simulink model "FSEA_Vehicle"  (R2026a)
settings: Solver=ode23tb  StopTime=5  FixedStep=.001  RelTol=1e-1
model workspace (MAT data in the model file):
  A_mu = 10
  B_reff = 8.386
  CONVERTER_DATA = [0  137.465208994  2.232; 0.1  137.065019157  2.075; 0.2  135.864449646  1.975; 0.3  135.664354728  1.846; 0.4  137.565256453  1.72; 0.5  140.366585312  1.564; 0.6  145.268910814  1.409; 0.7  152.872517717  1.254; 0.8  162.9773111  1.096; 0.81  164.27792807  1.08; 0.82  166.178829795  1.061; 0.83  167.979684062  1.043; 0.84  170.080680706  1.028; 0.85  172.781962105  1.012; 0.86  175.383196045  1.002; 0.87  179.585189333  1.002; 0.88  183.587087703  1.001; 0.89  189.890077635  0.998; 0.9  197.693779455  0.999; 0.92  215.902417037  1.001; 0.94  244.515990379  1.002]
  Cps = 2
  Cz = 7766.25
  DOWN_TABLE = [0  5  10  20  30; 0  5  10  20  30; 0  7.5  20  30  40; 0  7.5  20  30  40; 0  15  30  50  60; 0  15  30  50  60]
  DOWN_TH_BP = [0 5 40 50 90 100]
  D_reff = 0.25826
  EMAP = [-40  -44  -49  -53  -57  -61  -65  -70  -74  -78  -82; 215  117  85  66  44  29  10  -2  -13  -22  -32; 245  208  178  148  122  104  85  66  48  33  18; 264  260  241  219  193  167  152  133  119  96  85; 264  279  282  275  260  238  223  208  189  171  152; 267  290  293  297  290  275  260  256  234  212  193; 267  297  305  305  305  301  293  282  267  249  226; 267  301  308  312  319  323  319  316  297  279  253; 267  301  312  319  327  327  327  327  312  293  267; 267  301  312  319  327  334  334  334  319  305  275]
  F0z = [6086.4 4324.8]
  F_reff = 0.07394
  F_zmax = 10000
  F_zmin = 100
  F_zo = 4000
  Kz = 48000
  MF.f.mu_x = 1.2
  MF.f.mu_y = 0.935
  MF.f.Bx = 11.7
  MF.f.By = 8.86
  MF.f.Cx = 1.69
  MF.f.Cy = 1.19
  MF.f.Ex = 0.377
  MF.f.Ey = -1.21
  MF.f.Cxalpha = 1.09
  MF.f.Cykappa = 1.08
  MF.f.Bx1 = 12.4
  MF.f.Bx2 = -10.8
  MF.f.By1 = 6.46
  MF.f.By2 = 4.2
  MF.f.Sh = 0
  MF.f.Sv = 0
  MF.r.mu_x = 1.2
  MF.r.mu_y = 0.961
  MF.r.Bx = 11.1
  MF.r.By = 9.3
  MF.r.Cx = 1.69
  MF.r.Cy = 1.19
  MF.r.Ex = 0.362
  MF.r.Ey = -1.11
  MF.r.Cxalpha = 1.09
  MF.r.Cykappa = 1.08
  MF.r.Bx1 = 12.4
  MF.r.Bx2 = -10.8
  MF.r.By1 = 6.46
  MF.r.By2 = 4.2
  MF.r.Sh = 0
  MF.r.Sv = 0
  NCyl = 6
  NE_VEC = [800 1200 1600 2000 2400 2800 3200 3600 4000 4400 4800]
  Pstd = 101325
  Rair = 287
  SUS.Stiffness = 24000
  SUS.Damping.Constant = 1262
  SUS.Damping.Rebound = [4040 4950 2883 2043]
  SUS.Damping.Compression = [3600 3420 1863 1472]
  SUS.PistonSpeed = [0.05 0.1 0.3 0.6]
  SUS.UnsprungMass.Fr = 21.0693333333
  SUS.UnsprungMass.Rr = 21.0693333333
  TH_VEC = [0; 20; 30; 40; 50; 60; 70; 80; 90; 100]
  TWAITdn = 1.25
  TWAITup = 0.1
  Tin = [1  2; 2  2; 3  2; 4  2; 5  2; 6  0; 7  0; 8  0; 9  0; 10  0]
  Tstd = 293.15
  UP_TABLE = [7.5  25  40  50  60; 7.5  25  40  50  60; 15  35  50  60  70; 25  45  60  70  80; 40  70  90  100  110; 40  80  90  100  110]
  UP_TH_BP = [0 25 35 50 90 100]
  VEH.Mass = 1181
  VEH.StaticNormalFrontLoad.FR = 264.666666667
  VEH.StaticNormalFrontLoad.FL = 264.666666667
  VEH.StaticNormalRearLoad.RR = 322
  VEH.StaticNormalRearLoad.RL = 322
  VEH.WheelBase = 3.075
  VEH.FrontAxlePositionfromCG = 1.515
  VEH.RearAxlePositionfromCG = 1.504
  VEH.HeightCG = 0.134
  VEH.FrontalArea = 2.11
  VEH.DragCoefficient = 0.33
  VEH.NumberOfWheelsPerAxle = 2
  VEH.PitchMomentInertia = 1922.66666667
  VEH.RollMomentInertia = 432.333333333
  VEH.YawMomentInertia = 2066
  VEH.SteeringRatio = 18
  VEH.TrackWidth = 1.922
  VEH.SprungMass = 1096.72266667
  VEH.InitialLongPosition = 0
  VEH.InitialLatPosition = 0
  VEH.InitialVertPosition = 0
  VEH.InitialRollAngle = 0
  VEH.InitialPitchAngle = 0
  VEH.InitialYawAngle = 0
  VEH.InitialLongVel = 0
  VEH.InitialLatVel = 0
  VEH.InitialVertVel = 0
  VEH.InitialRollRate = 0
  VEH.InitialPitchRate = 0
  VEH.InitialYawRate = 0
  VEH.UnsprungMassRearAxle = 160
  VEH.UnsprungMassFrontAxle = 100
  V_o = 16.7
  V_xlow = 1
  Vd = 0.00346
  WH.Tire.Radius.Front = 0.384
  WH.Tire.Radius.Rear = 0.401
  WH.Tire.Sidewall = 0.245
  WH.Tire.RollingResistCoeff = 0.0103
  WH.Tire.Magic.B = 10
  WH.Tire.Magic.C = 1.9
  WH.Tire.Magic.D = 1
  WH.Tire.Magic.E = 0.97
  WH.Tire.Magic.Bx = 12
  WH.Tire.Magic.Cx = 1.9
  WH.Tire.Magic.Dx = 0.72
  WH.Tire.Magic.Ex = 0.95
  WH.Tire.Magic.By = 12
  WH.Tire.Magic.Cy = 1.3
  WH.Tire.Magic.Dy = 0.75
  WH.Tire.Magic.Ey = 0.2
  WH.Tire.Front.Ky = 40000
  WH.Tire.Rear.Ky = 40000
  WH.Tire.Kz = 320000
  WH.Tire.Damping = 100
  WH.Inertia = 1.00333333333
  WH.Mass = 11.4333333333
  WH.DampingCoefficient = 0.01
  WH.VelocityTol = 0.1
  a = 1.515
  alpha_max = 1.5
  alpha_min = -1.5
  b = 1.504
  c_zo = 209651
  epsilon = 0.1
  f_air = [0 0 0 0 0 0 0 0 0 0 0 0 ... (256 elements, 16x16)]
  f_co = [0 0 0 0 0 0 0 0 0 0 0 0 ... (256 elements, 16x16)]
  f_co2 = [0 0 0 0 0 0 0 0 0 0 0 0 ... (256 elements, 16x16)]
  f_eff = [352.135682859 352.135682859 320.724378192 303.655312657 295.930136708 291.240087194 291.240271258 291.240312459 291.240275452 291.240198499 291.240100781 291.240018769 ... (256 elements, 16x16)]
  f_fuel = [0 0 0 0 0 0 0 0 0 0 0 0 ... (256 elements, 16x16)]
  f_hc = [0 0 0 0 0 0 0 0 0 0 0 0 ... (256 elements, 16x16)]
  f_nox = [0 0 0 0 0 0 0 0 0 0 0 0 ... (256 elements, 16x16)]
  f_pm = [0  0  0  0  0  0  0  0  0  0  0  0  0  0  0  0; 0  0  0  0  0  0  0  0  0  0  0  0  0  0  0  0; 0  0  0  0  0  0  0  0  0  0  0  0  0  0  0  0; 0  0  0  0  0  0  0  0  0  0  0  0  0  0  0  0; 0  0  0  0  0  0  0  0  0  0  0  0  0  0  0  0; 0  0  0  0  0  0  0  0  0  0  0  0  0  0  0  0; 0  0  0  0  0  0  0  0  0  0  0  0  0  0  0  0; 0  0  0  0  0  0  0  0  0  0  0  0  0  0  0  0; 0  0  0  0  0  0  0  0  0  0  0  0  0  0  0  0; 0  0  0  0  0  0  0  0  0  0  0  0  0  0  0  0; 0  0  0  0  0  0  0  0  0  0  0  0  0  0  0  0; 0  0  0  0  0  0  0  0  0  0  0  0  0  0  0  0; 0  0  0  0  0  0  0  0  0  0  0  0  0  0  0  0; 0  0  0  0  0  0  0  0  0  0  0  0  0  0  0  0; 0  0  0  0  0  0  0  0  0  0  0  0  0  0  0  0; 0  0  0  0  0  0  0  0  0  0  0  0  0  0  0  0]
  f_susp_axl_bp = [1 2]
  f_susp_dz_bp = [-4 -0.14 -0.13 -0.12 -0.11 -0.1 -0.09 -0.08 -0.07 -0.06 -0.05 -0.04 -0.03 -0.02 -0.01 0 0.01 0.02 0.03 0.04 0.05 0.06 0.07 0.08 0.09 0.1 0.11 0.12 0.13 0.14 4]
  f_susp_dzdot_bp = [-4 -0.14 -0.13 -0.12 -0.11 -0.1 -0.09 -0.08 -0.07 -0.06 -0.05 -0.04 -0.03 -0.02 -0.01 0 0.01 0.02 0.03 0.04 0.05 0.06 0.07 0.08 0.09 0.1 0.11 0.12 0.13 0.14 4]
  f_susp_fmz = [-213379.591456 -28099.591456 -27619.591456 -27139.591456 -26659.591456 -26179.591456 -25699.591456 -25219.591456 -24739.591456 -24259.591456 -23779.591456 -23299.591456 ... (468968 elements, 31x31x61x2x4)]
  f_susp_geom = [-0.832564012244 0.043269987756 0.045538987756 0.047807987756 0.050076987756 0.052345987756 0.054614987756 0.056883987756 0.059152987756 0.061421987756 0.063690987756 0.065959987756 ... (11346 elements, 31x61x2x3)]
  f_susp_strgdelta_bp = [-0.523598775598 -0.506145483078 -0.488692190558 -0.471238898038 -0.453785605519 -0.436332312999 -0.418879020479 -0.401425727959 -0.383972435439 -0.366519142919 -0.349065850399 -0.331612557879 -0.314159265359 -0.296705972839 -0.279252680319 -0.261799387799 -0.244346095279 -0.226892802759 -0.209439510239 -0.191986217719 -0.174532925199 -0.157079632679 -0.13962634016 -0.12217304764 -0.10471975512 -0.0872664625997 -0.0698131700798 -0.0523598775598 -0.0349065850399 -0.0174532925199 0 0.0174532925199 0.0349065850399 0.0523598775598 0.0698131700798 0.0872664625997 0.10471975512 0.12217304764 0.13962634016 0.157079632679 0.174532925199 0.191986217719 0.209439510239 0.226892802759 0.244346095279 0.261799387799 0.279252680319 0.296705972839 0.314159265359 0.331612557879 0.349065850399 0.366519142919 0.383972435439 0.401425727959 0.418879020479 0.436332312999 0.453785605519 0.471238898038 0.488692190558 0.506145483078 0.523598775598]
  f_tbrake = [0 76.8593923996 105.140482948 131.533638111 157.926793274 176.658631717 176.65727296 176.656856686 176.656879077 176.657093756 176.657404516 176.65772406 ... (256 elements, 16x16)]
  f_tbrake_n_bpt = [0 649.519052838 912.419621844 1175.32019085 1438.22075986 1701.12132886 1964.02189787 2226.92246687 2489.82303588 2752.72360489 3015.62417389 3278.5247429 3541.4253119 3804.32588091 4067.22644992 4330.12701892]
  f_tbrake_t_bpt = [0 34.6410161514 61.0341713143 87.4273264773 113.82048164 140.213636803 166.606791966 192.999947129 219.393102292 245.786257455 272.179412618 298.572567781 324.965722944 351.358878107 377.75203327 404.145188433]
  f_texh = [766.752464599 766.752464599 786.17542386 801.679939032 884.591982581 910.574397722 910.571871054 910.570774534 910.570601632 910.570821151 910.571247242 910.571639815 ... (256 elements, 16x16)]
  f_twc_eff_co = [0.17 0.25 0.45 0.99 0.99 0.99 0.99]
  f_twc_eff_hc = [0.21 0.375 0.75 0.98 0.98 0.98 0.98]
  f_twc_eff_lam = [0.909090909 0.944055944 0.979020979 1 1.013986014 1.048951049 1.083916084]
  f_twc_eff_nox = [0.98 0.98 0.98 0.97 0.05 0.02 0]
  h = 0.134
  k_z = 50
  kappa_max = 1.5
  kappa_min = -1.5
  lam_Cx = 1
  lam_Cy = 1
  lam_Cz = 1
  lam_Ex = 1
  lam_Ey = 1
  lam_F_zo = 1
  lam_Hx = 1
  lam_Hy = 1
  lam_Kxkappa = 1
  lam_Kyalpha = 1
  lam_Kygamma = 1
  lam_Kzgamma = 1
  lam_Mr = 1
  lam_Mx = 1
  lam_My = 1
  lam_S = 1
  lam_VMx = 1
  lam_Vx = 1
  lam_Vy = 1
  lam_Vykappa = 1
  lam_muV = 0
  lam_mux = 1
  lam_muy = 1
  lam_t = 1
  lam_xalpha = 1
  lam_ykappa = 1
  numWheel = 4
  p_Cx1 = 1.579
  p_Cy1 = 1.3332
  p_Dx1 = 1.0422
  p_Dx2 = -0.08285
  p_Dx3 = 0
  p_Dy1 = 0.8784
  p_Dy2 = -0.06445
  p_Dy3 = 0
  p_Ex1 = 0.11185
  p_Ex2 = 0.3127
  p_Ex3 = 0
  p_Ex4 = 0.001603
  p_Ey1 = -0.8227
  p_Ey2 = -0.6062
  p_Ey3 = 0.09825
  p_Ey4 = -6.546
  p_Ey5 = 0
  p_Fz1 = 0.7098
  p_Hx1 = 0.00021585
  p_Hx2 = 0.0011538
  p_Hy1 = -0.0018043
  p_Hy2 = 0.003518
  p_Kx1 = 21.69
  p_Kx2 = 13.774
  p_Kx3 = -0.4119
  p_Ky1 = -15.314
  p_Ky2 = 1.7044
  p_Ky3 = 0.36986
  p_Ky4 = 1.9896
  p_Ky5 = 0
  p_Ky6 = -0.9004
  p_Ky7 = -0.2328
  p_Vx1 = 1.5973e-05
  p_Vx2 = 0.0001043
  p_Vy1 = -0.006642
  p_Vy2 = 0.03597
  p_Vy3 = -0.1621
  p_Vy4 = -0.4908
  p_pmx1 = 0
  p_px1 = -0.3489
  p_px2 = 0.382
  p_px3 = -0.09634
  p_px4 = 0.06447
  p_py1 = -0.6249
  p_py2 = -0.06535
  p_py3 = -0.1668
  p_py4 = 0.2834
  p_py5 = 0
  path.ISO3888p2.x = [0 2 12 25.5 36.5 49 61]
  path.ISO3888p2.y = [0 0 0 3.725 3.725 0 0]
  path.ISO3888p2.ylb = [1.225 1.225 1.225 4.725 4.725 1.5 1.5]
  path.ISO3888p2.yrb = [-1.225 -1.225 -1.225 2.225 2.225 -1.5 -1.5]
  path.CUSC.x = [10.668 21.336 36.576 54.864 73.152]
  path.CUSC.y = [0 0 5.1816 0 0]
  path.CUSC.ylb = [1.2192 1.2192 7.0104 1.8288 1.8288]
  path.CUSC.yrb = [-1.2192 -1.2192 3.3528 -1.8288 -1.8288]
  pio = 220000
  q_Fcx = 0
  q_Fz2 = 15.4
  q_Fzy = 0
  q_reo = 0.9974
  q_sx1 = -0.007764
  q_sx10 = 0.2824
  q_sx11 = 5.349
  q_sx12 = 0
  q_sx13 = 0
  q_sx14 = 0
  q_sx2 = 1.1915
  q_sx3 = 0.013948
  q_sx4 = 4.912
  q_sx5 = 1.02
  q_sx6 = 22.83
  q_sx7 = 0.7104
  q_sx8 = -0.023393
  q_sx9 = 0.6581
  q_sy1 = 0.00702
  q_sy2 = 0
  q_sy3 = 0.001515
  q_sy4 = 8.514e-05
  q_sy5 = 0
  q_sy6 = 0
  q_sy7 = 0.9008
  q_sy8 = -0.4089
  q_v1 = 0.0007742
  q_v2 = 0.04667
  r_Bx1 = 12.531
  r_Bx2 = 9.532
  r_Bx3 = 0
  r_By1 = 10.615
  r_By2 = 7.705
  r_By3 = 3.433e-06
  r_By4 = 0
  r_Cx1 = 1.019
  r_Cy1 = 1.0585
  r_Ex1 = -0.4487
  r_Ex2 = -0.4726
  r_Ey1 = 0.3132
  r_Ey2 = 7.63e-06
  r_Hx1 = 0.0002374
  r_Hy1 = 0.011646
  r_Hy2 = 7.63e-06
  r_Vy1 = 0.05654
  r_Vy2 = 7.63e-06
  r_Vy3 = 0
  r_Vy4 = 99.9
  r_Vy5 = 2
  r_Vy6 = 15.814
  r_o = 0.3135
  reqTmaxT = [nan  nan  nan  nan  nan  nan  nan  nan; 0.285774810084  0.209689533834  0.17164689571  0.133604257585  0.0955616194602  nan  nan  nan; 0.647179872268  0.495009319769  0.41892404352  0.342838767271  0.266753491021  0.152625576647  nan  nan; nan  0.780329105704  0.66620119133  0.552073276956  0.437945362582  0.266753491021  0.152625576647  0.0955616194602; nan  nan  0.913478339141  0.761307786642  0.609137234143  0.380881405395  0.228710852897  0.152625576647; nan  nan  nan  0.970542296328  0.780329105704  0.495009319769  0.304796129146  0.209689533834; nan  nan  nan  nan  0.951520977265  0.609137234143  0.380881405395  0.266753491021; nan  nan  nan  nan  nan  0.723265148517  0.456966681645  0.323817448208; nan  nan  nan  nan  nan  0.837393062891  0.533051957894  0.380881405395; nan  nan  nan  nan  nan  0.951520977265  0.609137234143  0.437945362582; nan  nan  nan  nan  nan  nan  0.685222510393  0.495009319769; nan  nan  nan  nan  nan  nan  0.761307786642  0.552073276956; nan  nan  nan  nan  nan  nan  0.837393062891  0.609137234143; nan  nan  nan  nan  nan  nan  0.913478339141  0.66620119133; nan  nan  nan  nan  nan  nan  0.98956361539  0.723265148517; nan  nan  nan  nan  nan  nan  nan  0.780329105704; nan  nan  nan  nan  nan  nan  nan  0.837393062891; nan  nan  nan  nan  nan  nan  nan  0.894457020078; nan  nan  nan  nan  nan  nan  nan  0.951520977265; nan  nan  nan  nan  nan  nan  nan  nan; nan  nan  nan  nan  nan  nan  nan  nan]
  vehSpd = [0 2.77777777778 5.55555555556 8.33333333333 11.1111111111 13.8888888889 16.6666666667 19.4444444444 22.2222222222 25 27.7777777778 30.5555555556 33.3333333333 36.1111111111 38.8888888889 41.6666666667 44.4444444444 47.2222222222 50 52.7777777778 55.5555555556]
  vehWidth = 2
  w = 1
undefined symbols (not defined in the file or in its folder): InertFrm
libraries: sharedtransform x6, vehdynlibtirecommon x2, vehdynlibtire x2, autolibutils x2, autolibshared x2
(part 1 of 4)
settings Model: DataDictionary=PassVeh7DOF.sldd  ModifiedByFormat=The MathWorks, Inc.  SimulationMode=accelerator  Creator=The MathWorks, Inc.  LastModifiedBy=The MathWorks, Inc.
settings SolverCC: SolverJacobianMethodControl=FullPerturbation  ZeroCrossAlgorithm=Adaptive  DecoupledContinuousIntegration=on
settings DebuggingCC: ArtificialAlgebraicLoopMsg=none  MaskedZcDiagnostic=none  IgnoredZcDiagnostic=none  SignalLabelMismatchMsg=warning
settings ModelReferenceCC: ModelReferenceMinAlgLoopOccurrences=on

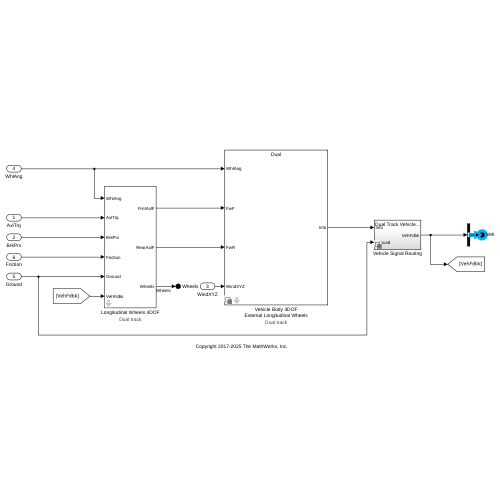
[thumbnail: Simulink's stored preview of the top-level diagram]
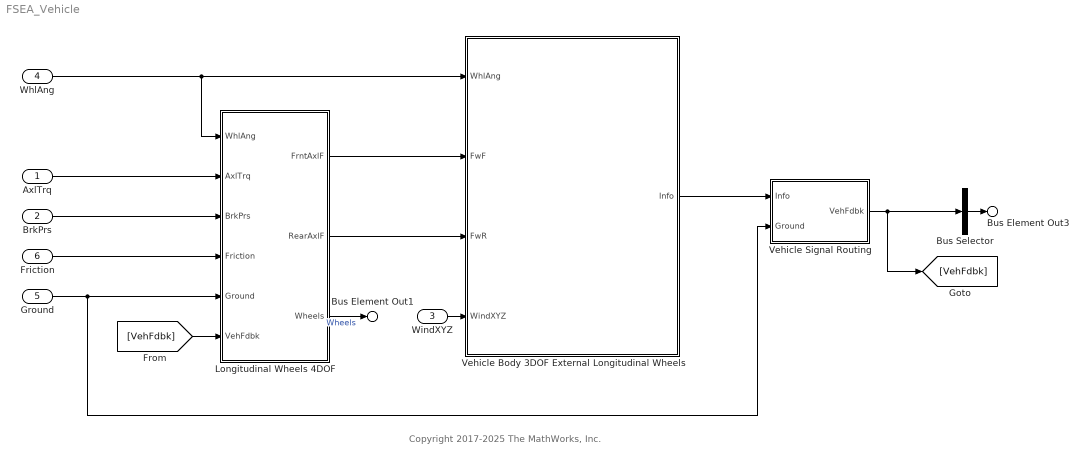
== system FSEA_Vehicle ==
  note: Copyright 2017-2025 The MathWorks, Inc.
  AxlTrq : Inport  Unit=N*m  PortDimensions=4
  BrkPrs : Inport  Port=2  Unit=Pa  PortDimensions=4
  WindXYZ : Inport  Port=3  PortDimensions=3
  WhlAng : Inport  Port=4  Unit=rad  PortDimensions=4
  Ground : Inport  Port=5  Unit=m  PortDimensions=4
  Friction : Inport  Port=6  Unit=1  PortDimensions=4
  Bus Selector : BusSelector  OutputSignals=InertFrm,BdyFrm  OutputAsBus=on
  Longitudinal Wheels 4DOF : Subsystem  VariantControl=1  mask{wheelMode=Dual track}
      mask prompts: wheelMode "Wheel mode:"
      settings: AttributesFormatString=%<wheelMode>
      mask TypeOptions wheelMode: Single track (bicycle) | Dual track
      mask Callback wheelMode:
      | switch get_param(gcb,'wheelMode')
      |     case 'Single track (bicycle)'
      |         set_param([bdroot '/Longitudinal Wheels 4DOF/Velocity and Vertical Load'],'OverrideUsingVariant','0')
      |         set_param([bdroot '/Longitudinal Wheels 4DOF/Axle Forces'],'OverrideUsingVariant','0')
      |     case 'Dual track'
      |         set_param([bdroot '/Longitudinal Wheels 4DOF/Velocity and Vertical Load'],'OverrideUsingVariant','1')
      |         set_param([bdroot '/Longitudinal Wheels 4DOF/Axle Forces'],'OverrideUsingVariant','1')
      |     otherwise
      |         set_param([bdroot '/Longitudinal Wheels 4DOF/Velocity and Vertical Load'],'OverrideUsingVariant','0')
      |         set_param([bdroot '/Longitudinal Wheels 4DOF/Axle Forces'],'OverrideUsingVariant','0')
      | end
  Vehicle Body 3DOF External Longitudinal Wheels : Subsystem  Variant=on  VariantControlMode=label  VariantControl=Variant1  LabelModeActiveChoice=1  mask(Example 3DOF vehicle model){trackMode=Dual track}
      mask prompts: trackMode "Vehicle Mode:"
      mask help: Select the variant of the 3DOF vehicle model. The wheel subsystem will be automatically configured accordingly.
      settings: AttributesFormatString=%<trackMode>
      mask TypeOptions trackMode: Single track (bicycle) | Dual track
      mask Callback trackMode:
      | switch get_param(gcb,'trackMode')
      |     case 'Single track (bicycle)'
      |         set_param([bdroot '/Vehicle Body 3DOF' newline 'External Longitudinal Wheels'],'OverrideUsingVariant','0')
      |         set_param([bdroot '/Longitudinal Wheels 4DOF'],'wheelMode','Single track (bicycle)')
      |         set_param([bdroot '/Longitudinal Wheels 4DOF/Velocity and Vertical Load'],'OverrideUsingVariant','0')
      |         set_param([bdroot '/Longitudinal Wheels 4DOF/Axle Forces'],'OverrideUsingVariant','0')
      |         set_param([bdroot '/Vehicle Signal Routing'],'OverrideUsingVariant','0')
      |     case 'Dual track'
      |         set_param([bdroot '/Vehicle Body 3DOF' newline 'External Longitudinal Wheels'],'OverrideUsingVariant','1')
      |         set_param([bdroot '/Longitudinal Wheels 4DOF'],'wheelMode','Dual track')
      |         set_param([bdroot '/Longitudinal Wheels 4DOF/Velocity and Vertical Load'],'OverrideUsingVariant','1')
      |         set_param([bdroot '/Longitudinal Wheels 4DOF/Axle Forces'],'OverrideUsingVariant','1')
      |         set_param([bdroot '/Vehicle Signal Routing'],'OverrideUsingVariant','1')
      |     otherwise
      |         set_param([bdroot '/Wheels and Brakes'],'OverrideUsingVariant','0')
      |         set_param([bdroot '/Longitudinal Wheels 4DOF'],'wheelMode','Single track (bicycle)')
      |         set_param([bdroot '/Longitudinal Wheels 4DOF/Velocity and Vertical Load'],'OverrideUsingVariant','0')
      |         set_param([bdroot '/Longitudinal Wheels 4DOF/Axle Forces'],'OverrideUsingVariant','0')
      |         set_param([bdroot '/Vehicle Signal Routing'],'OverrideUsingVariant','0')
      | end
  Vehicle Signal Routing : Subsystem  Variant=on  VariantControlMode=label  LabelModeActiveChoice=1
  Bus Element Out3 : Outport  PortName=Veh
  Bus Element Out1 : Outport  Port=2  PortName=Wheels
  wires:
  WindXYZ/1 -> Vehicle Body 3DOF External Longitudinal Wheels/4(WindXYZ)
  Friction/1 -> Longitudinal Wheels 4DOF/4(Friction)
  Longitudinal Wheels 4DOF/1(FrntAxlF) -> Vehicle Body 3DOF External Longitudinal Wheels/2("FwF ")
  Longitudinal Wheels 4DOF/2(RearAxlF) -> Vehicle Body 3DOF External Longitudinal Wheels/3("FwR ")
  Ground/1 -> Longitudinal Wheels 4DOF/5(Ground), Vehicle Signal Routing/2(Ground)
  Longitudinal Wheels 4DOF/3(Wheels) -> Bus Element Out1/1  "Wheels"
  Bus Selector/1 -> Bus Element Out3/1
  AxlTrq/1 -> Longitudinal Wheels 4DOF/2(AxlTrq)
  BrkPrs/1 -> Longitudinal Wheels 4DOF/3(BrkPrs)
  WhlAng/1 -> Vehicle Body 3DOF External Longitudinal Wheels/1(WhlAng), Longitudinal Wheels 4DOF/1(WhlAng)
  [VehFdbk] -> Longitudinal Wheels 4DOF/6(VehFdbk)
  Vehicle Body 3DOF External Longitudinal Wheels/1(" Info") -> Vehicle Signal Routing/1(Info)
  Vehicle Signal Routing/1(VehFdbk) -> Bus Selector/1, [VehFdbk]
